simulink model "p2_1_neuron"  (R2025b)
settings: Solver=ode45  StartTime=0.0  StopTime=40  MaxStep=0.01  RelTol=1e-6
undefined symbols (not defined in the file or in its folder): np
settings Model: Creator=maria  LastModifiedBy=maria

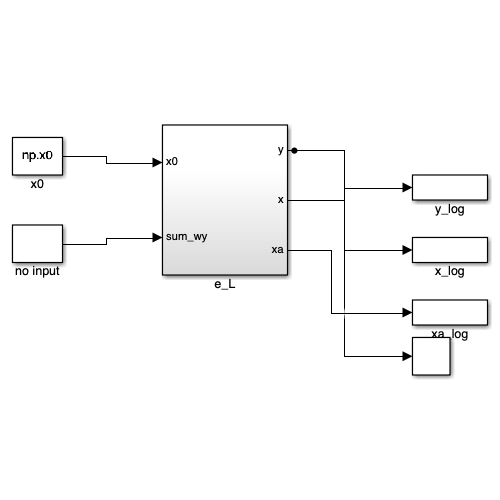
[thumbnail: Simulink's stored preview of the top-level diagram]
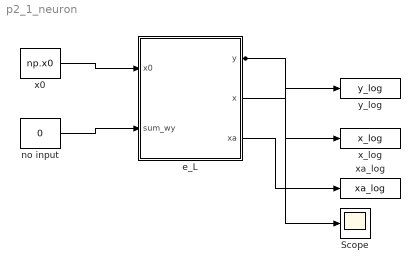
== system p2_1_neuron ==
  Scope : Scope
  e_L : Subsystem
  no input : Constant  Value=0
  x0 : Constant  Value=np.x0
  x_log : ToWorkspace  VariableName=x_log  SaveFormat=Timeseries  SampleTime=-1
  xa_log : ToWorkspace  VariableName=xa_log  SaveFormat=Timeseries  SampleTime=-1
  y_log : ToWorkspace  VariableName=y_log  SaveFormat=Timeseries  SampleTime=-1
  wires:
  e_L/1(y) -> y_log/1, Scope/1
  e_L/2(x) -> x_log/1
  e_L/3(xa) -> xa_log/1
  x0/1 -> e_L/1(x0)
  no input/1 -> e_L/2(sum_wy)

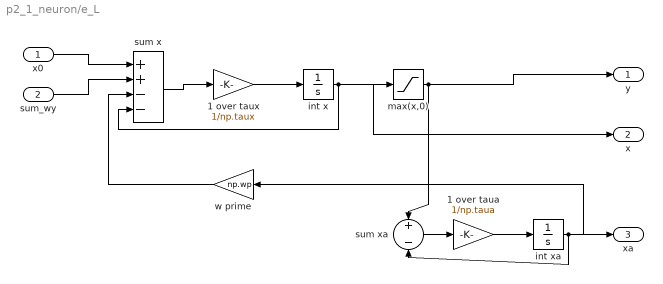
== system p2_1_neuron/e_L ==
  x0 : Inport
  sum_wy : Inport  Port=2
  1 over taua : Gain  Gain=1/np.taua
  1 over taux : Gain  Gain=1/np.taux
  int x : Integrator
  int xa : Integrator
  max(x,0) : Saturate  UpperLimit=inf  LowerLimit=0
  sum x : Sum  Inputs=++--
  sum xa : Sum  Inputs=+-
  w prime : Gain  Gain=np.wp
  y : Outport
  x : Outport  Port=2
  xa : Outport  Port=3
  wires:
  x0/1 -> sum x/1
  sum_wy/1 -> sum x/2
  w prime/1 -> sum x/3
  int x/1 -> sum x/4, max(x,0)/1, x/1
  sum x/1 -> 1 over taux/1
  1 over taux/1 -> int x/1
  max(x,0)/1 -> y/1, sum xa/1
  int xa/1 -> sum xa/2, xa/1, w prime/1
  sum xa/1 -> 1 over taua/1
  1 over taua/1 -> int xa/1
